simulink model "GaN_Fig5_Clamp_Analog_State"  (R2022b)
settings: Solver=ode15s  StartTime=0.0  StopTime=3e-6  MaxStep=5e-10  RelTol=1e-7  AbsTol=1e-9
model workspace (MAT data in the model file):
  btb_blocking_negative = [0 1e-10 2e-10 3e-10 4e-10 5e-10 6e-10 7e-10 8e-10 9e-10 1e-09 1.1e-09 ... (60002 elements, 30001x2)]
  btb_blocking_positive = [0 1e-10 2e-10 3e-10 4e-10 5e-10 6e-10 7e-10 8e-10 9e-10 1e-09 1.1e-09 ... (60002 elements, 30001x2)]
  btb_improved_negative = [0 1e-10 2e-10 3e-10 4e-10 5e-10 6e-10 7e-10 8e-10 9e-10 1e-09 1.1e-09 ... (60002 elements, 30001x2)]
  btb_improved_positive = [0 1e-10 2e-10 3e-10 4e-10 5e-10 6e-10 7e-10 8e-10 9e-10 1e-09 1.1e-09 ... (60002 elements, 30001x2)]
  dv_blocking_negative = [0 1e-10 2e-10 3e-10 4e-10 5e-10 6e-10 7e-10 8e-10 9e-10 1e-09 1.1e-09 ... (60002 elements, 30001x2)]
  dv_blocking_positive = [0 1e-10 2e-10 3e-10 4e-10 5e-10 6e-10 7e-10 8e-10 9e-10 1e-09 1.1e-09 ... (60002 elements, 30001x2)]
  dv_improved_negative = [0 1e-10 2e-10 3e-10 4e-10 5e-10 6e-10 7e-10 8e-10 9e-10 1e-09 1.1e-09 ... (60002 elements, 30001x2)]
  dv_improved_positive = [0 1e-10 2e-10 3e-10 4e-10 5e-10 6e-10 7e-10 8e-10 9e-10 1e-09 1.1e-09 ... (60002 elements, 30001x2)]
  gb_blocking_negative = [0 1e-10 2e-10 3e-10 4e-10 5e-10 6e-10 7e-10 8e-10 9e-10 1e-09 1.1e-09 ... (60002 elements, 30001x2)]
  gb_blocking_positive = [0 1e-10 2e-10 3e-10 4e-10 5e-10 6e-10 7e-10 8e-10 9e-10 1e-09 1.1e-09 ... (60002 elements, 30001x2)]
  gb_improved_negative = [0 1e-10 2e-10 3e-10 4e-10 5e-10 6e-10 7e-10 8e-10 9e-10 1e-09 1.1e-09 ... (60002 elements, 30001x2)]
  gb_improved_positive = [0 1e-10 2e-10 3e-10 4e-10 5e-10 6e-10 7e-10 8e-10 9e-10 1e-09 1.1e-09 ... (60002 elements, 30001x2)]
  v_blocking_negative = [0 1e-10 2e-10 3e-10 4e-10 5e-10 6e-10 7e-10 8e-10 9e-10 1e-09 1.1e-09 ... (60002 elements, 30001x2)]
  v_blocking_positive = [0 1e-10 2e-10 3e-10 4e-10 5e-10 6e-10 7e-10 8e-10 9e-10 1e-09 1.1e-09 ... (60002 elements, 30001x2)]
  v_improved_negative = [0 1e-10 2e-10 3e-10 4e-10 5e-10 6e-10 7e-10 8e-10 9e-10 1e-09 1.1e-09 ... (60002 elements, 30001x2)]
  v_improved_positive = [0 1e-10 2e-10 3e-10 4e-10 5e-10 6e-10 7e-10 8e-10 9e-10 1e-09 1.1e-09 ... (60002 elements, 30001x2)]
settings Model: Creator=Greatlovers  LastModifiedBy=Greatlovers

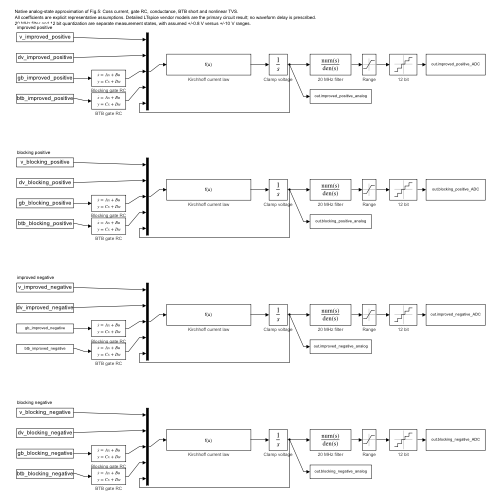
[thumbnail: Simulink's stored preview of the top-level diagram]
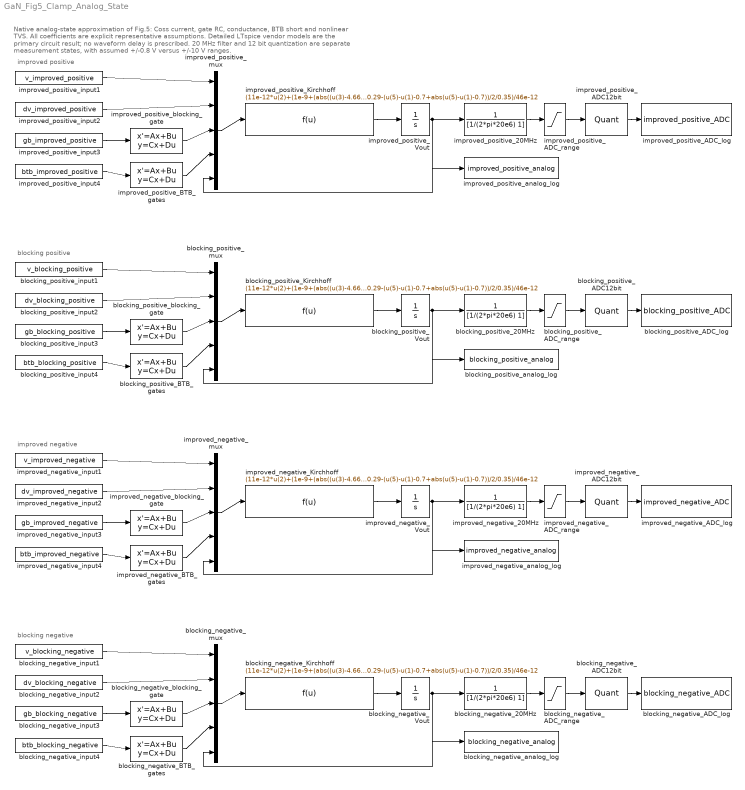
== system GaN_Fig5_Clamp_Analog_State ==
  note: improved positive
  note: blocking positive
  note: improved negative
  note: blocking negative
  note: Native analog-state approximation of Fig.5: Coss current, gate RC, conductance, BTB short and nonlinear TVS.
      | All coefficients are explicit representative assumptions. Detailed LTspice vendor models are the primary circuit result; no waveform delay is prescribed.
      | 20 MHz filter and 12 bit quantization are separate measurement states, with assumed +/-0.8 V versus +/-10 V ranges.
  blocking_negative_20MHz : TransferFcn  Numerator=1  Denominator=[1/(2*pi*20e6) 1]
      settings: AttributesFormatString=20 MHz filter
  blocking_negative_ADC12bit : Quantizer  QuantizationInterval=0.0048828125
      settings: AttributesFormatString=12 bit
  blocking_negative_ADC_log : ToWorkspace  VariableName=blocking_negative_ADC  SaveFormat=Timeseries  SampleTime=-1
  blocking_negative_ADC_range : Saturate  UpperLimit=10  LowerLimit=-10
      settings: AttributesFormatString=Range
  blocking_negative_BTB_gates : StateSpace  A=-1/2.6e-9  B=1/2.6e-9  D=0  InitialCondition=0
      settings: AttributesFormatString=BTB gate RC
  blocking_negative_Kirchhoff : Fcn  Expr=(11e-12*u(2)+(1e-9+(abs((u(3)-4.662)/5.338)-abs((u(3)-4.662)/5.338-1)+1)/2/11)*(u(1)-u(5))-(abs((u(4)-0.6118)/3.8882)-abs((u(4)-0.6118)/3.8882-1)+1)/2/0.122*u(5)-u(5)/1e6-((u(5)-8+abs(u(5)-8))/2-(-u(5)-8+abs(-u(5)-8))/2)/0.29-(u(5)-u(1)-0.7+abs(u(5)-u(1)-0.7))/2/0.35)/46e-12
      settings: AttributesFormatString=Kirchhoff current law
  blocking_negative_Vout : Integrator
      settings: AttributesFormatString=Clamp voltage
  blocking_negative_analog_log : ToWorkspace  VariableName=blocking_negative_analog  SaveFormat=Timeseries  SampleTime=-1
  blocking_negative_blocking_gate : StateSpace  A=-1/1.88e-9  B=1/1.88e-9  D=0  InitialCondition=0
      settings: AttributesFormatString=Blocking gate RC
  blocking_negative_input1 : FromWorkspace  VariableName=v_blocking_negative
  blocking_negative_input2 : FromWorkspace  VariableName=dv_blocking_negative
  blocking_negative_input3 : FromWorkspace  VariableName=gb_blocking_negative
  blocking_negative_input4 : FromWorkspace  VariableName=btb_blocking_negative
  blocking_negative_mux : Mux  Inputs=5
  blocking_positive_20MHz : TransferFcn  Numerator=1  Denominator=[1/(2*pi*20e6) 1]
      settings: AttributesFormatString=20 MHz filter
  blocking_positive_ADC12bit : Quantizer  QuantizationInterval=0.0048828125
      settings: AttributesFormatString=12 bit
  blocking_positive_ADC_log : ToWorkspace  VariableName=blocking_positive_ADC  SaveFormat=Timeseries  SampleTime=-1
  blocking_positive_ADC_range : Saturate  UpperLimit=10  LowerLimit=-10
      settings: AttributesFormatString=Range
  blocking_positive_BTB_gates : StateSpace  A=-1/2.6e-9  B=1/2.6e-9  D=0  InitialCondition=0
      settings: AttributesFormatString=BTB gate RC
  blocking_positive_Kirchhoff : Fcn  Expr=(11e-12*u(2)+(1e-9+(abs((u(3)-4.662)/5.338)-abs((u(3)-4.662)/5.338-1)+1)/2/11)*(u(1)-u(5))-(abs((u(4)-0.6118)/3.8882)-abs((u(4)-0.6118)/3.8882-1)+1)/2/0.122*u(5)-u(5)/1e6-((u(5)-8+abs(u(5)-8))/2-(-u(5)-8+abs(-u(5)-8))/2)/0.29-(u(5)-u(1)-0.7+abs(u(5)-u(1)-0.7))/2/0.35)/46e-12
      settings: AttributesFormatString=Kirchhoff current law
  blocking_positive_Vout : Integrator
      settings: AttributesFormatString=Clamp voltage
  blocking_positive_analog_log : ToWorkspace  VariableName=blocking_positive_analog  SaveFormat=Timeseries  SampleTime=-1
  blocking_positive_blocking_gate : StateSpace  A=-1/1.88e-9  B=1/1.88e-9  D=0  InitialCondition=0
      settings: AttributesFormatString=Blocking gate RC
  blocking_positive_input1 : FromWorkspace  VariableName=v_blocking_positive
  blocking_positive_input2 : FromWorkspace  VariableName=dv_blocking_positive
  blocking_positive_input3 : FromWorkspace  VariableName=gb_blocking_positive
  blocking_positive_input4 : FromWorkspace  VariableName=btb_blocking_positive
  blocking_positive_mux : Mux  Inputs=5
  improved_negative_20MHz : TransferFcn  Numerator=1  Denominator=[1/(2*pi*20e6) 1]
      settings: AttributesFormatString=20 MHz filter
  improved_negative_ADC12bit : Quantizer  QuantizationInterval=0.00039062500000000002
      settings: AttributesFormatString=12 bit
  improved_negative_ADC_log : ToWorkspace  VariableName=improved_negative_ADC  SaveFormat=Timeseries  SampleTime=-1
  improved_negative_ADC_range : Saturate  UpperLimit=0.8  LowerLimit=-0.8
      settings: AttributesFormatString=Range
  improved_negative_BTB_gates : StateSpace  A=-1/2.6e-9  B=1/2.6e-9  D=0  InitialCondition=4.5
      settings: AttributesFormatString=BTB gate RC
  improved_negative_Kirchhoff : Fcn  Expr=(11e-12*u(2)+(1e-9+(abs((u(3)-4.662)/5.338)-abs((u(3)-4.662)/5.338-1)+1)/2/11)*(u(1)-u(5))-(abs((u(4)-0.6118)/3.8882)-abs((u(4)-0.6118)/3.8882-1)+1)/2/0.122*u(5)-u(5)/1e6-((u(5)-8+abs(u(5)-8))/2-(-u(5)-8+abs(-u(5)-8))/2)/0.29-(u(5)-u(1)-0.7+abs(u(5)-u(1)-0.7))/2/0.35)/46e-12
      settings: AttributesFormatString=Kirchhoff current law
  improved_negative_Vout : Integrator
      settings: AttributesFormatString=Clamp voltage
  improved_negative_analog_log : ToWorkspace  VariableName=improved_negative_analog  SaveFormat=Timeseries  SampleTime=-1
  improved_negative_blocking_gate : StateSpace  A=-1/1.88e-9  B=1/1.88e-9  D=0  InitialCondition=0
      settings: AttributesFormatString=Blocking gate RC
  improved_negative_input1 : FromWorkspace  VariableName=v_improved_negative
  improved_negative_input2 : FromWorkspace  VariableName=dv_improved_negative
  improved_negative_input3 : FromWorkspace  VariableName=gb_improved_negative
  improved_negative_input4 : FromWorkspace  VariableName=btb_improved_negative
  improved_negative_mux : Mux  Inputs=5
  improved_positive_20MHz : TransferFcn  Numerator=1  Denominator=[1/(2*pi*20e6) 1]
      settings: AttributesFormatString=20 MHz filter
  improved_positive_ADC12bit : Quantizer  QuantizationInterval=0.00039062500000000002
      settings: AttributesFormatString=12 bit
  improved_positive_ADC_log : ToWorkspace  VariableName=improved_positive_ADC  SaveFormat=Timeseries  SampleTime=-1
  improved_positive_ADC_range : Saturate  UpperLimit=0.8  LowerLimit=-0.8
      settings: AttributesFormatString=Range
  improved_positive_BTB_gates : StateSpace  A=-1/2.6e-9  B=1/2.6e-9  D=0  InitialCondition=4.5
      settings: AttributesFormatString=BTB gate RC
  improved_positive_Kirchhoff : Fcn  Expr=(11e-12*u(2)+(1e-9+(abs((u(3)-4.662)/5.338)-abs((u(3)-4.662)/5.338-1)+1)/2/11)*(u(1)-u(5))-(abs((u(4)-0.6118)/3.8882)-abs((u(4)-0.6118)/3.8882-1)+1)/2/0.122*u(5)-u(5)/1e6-((u(5)-8+abs(u(5)-8))/2-(-u(5)-8+abs(-u(5)-8))/2)/0.29-(u(5)-u(1)-0.7+abs(u(5)-u(1)-0.7))/2/0.35)/46e-12
      settings: AttributesFormatString=Kirchhoff current law
  improved_positive_Vout : Integrator
      settings: AttributesFormatString=Clamp voltage
  improved_positive_analog_log : ToWorkspace  VariableName=improved_positive_analog  SaveFormat=Timeseries  SampleTime=-1
  improved_positive_blocking_gate : StateSpace  A=-1/1.88e-9  B=1/1.88e-9  D=0  InitialCondition=0
      settings: AttributesFormatString=Blocking gate RC
  improved_positive_input1 : FromWorkspace  VariableName=v_improved_positive
  improved_positive_input2 : FromWorkspace  VariableName=dv_improved_positive
  improved_positive_input3 : FromWorkspace  VariableName=gb_improved_positive
  improved_positive_input4 : FromWorkspace  VariableName=btb_improved_positive
  improved_positive_mux : Mux  Inputs=5
  wires:
  improved_positive_input1/1 -> improved_positive_mux/1
  improved_positive_input2/1 -> improved_positive_mux/2
  improved_positive_input3/1 -> improved_positive_blocking_gate/1
  improved_positive_input4/1 -> improved_positive_BTB_gates/1
  improved_positive_blocking_gate/1 -> improved_positive_mux/3
  improved_positive_BTB_gates/1 -> improved_positive_mux/4
  improved_positive_mux/1 -> improved_positive_Kirchhoff/1
  improved_positive_Kirchhoff/1 -> improved_positive_Vout/1
  improved_positive_Vout/1 -> improved_positive_mux/5, improved_positive_20MHz/1, improved_positive_analog_log/1
  improved_positive_20MHz/1 -> improved_positive_ADC_range/1
  improved_positive_ADC_range/1 -> improved_positive_ADC12bit/1
  improved_positive_ADC12bit/1 -> improved_positive_ADC_log/1
  blocking_positive_input1/1 -> blocking_positive_mux/1
  blocking_positive_input2/1 -> blocking_positive_mux/2
  blocking_positive_input3/1 -> blocking_positive_blocking_gate/1
  blocking_positive_input4/1 -> blocking_positive_BTB_gates/1
  blocking_positive_blocking_gate/1 -> blocking_positive_mux/3
  blocking_positive_BTB_gates/1 -> blocking_positive_mux/4
  blocking_positive_mux/1 -> blocking_positive_Kirchhoff/1
  blocking_positive_Kirchhoff/1 -> blocking_positive_Vout/1
  blocking_positive_Vout/1 -> blocking_positive_mux/5, blocking_positive_20MHz/1, blocking_positive_analog_log/1
  blocking_positive_20MHz/1 -> blocking_positive_ADC_range/1
  blocking_positive_ADC_range/1 -> blocking_positive_ADC12bit/1
  blocking_positive_ADC12bit/1 -> blocking_positive_ADC_log/1
  improved_negative_input1/1 -> improved_negative_mux/1
  improved_negative_input2/1 -> improved_negative_mux/2
  improved_negative_input3/1 -> improved_negative_blocking_gate/1
  improved_negative_input4/1 -> improved_negative_BTB_gates/1
  improved_negative_blocking_gate/1 -> improved_negative_mux/3
  improved_negative_BTB_gates/1 -> improved_negative_mux/4
  improved_negative_mux/1 -> improved_negative_Kirchhoff/1
  improved_negative_Kirchhoff/1 -> improved_negative_Vout/1
  improved_negative_Vout/1 -> improved_negative_mux/5, improved_negative_20MHz/1, improved_negative_analog_log/1
  improved_negative_20MHz/1 -> improved_negative_ADC_range/1
  improved_negative_ADC_range/1 -> improved_negative_ADC12bit/1
  improved_negative_ADC12bit/1 -> improved_negative_ADC_log/1
  blocking_negative_input1/1 -> blocking_negative_mux/1
  blocking_negative_input2/1 -> blocking_negative_mux/2
  blocking_negative_input3/1 -> blocking_negative_blocking_gate/1
  blocking_negative_input4/1 -> blocking_negative_BTB_gates/1
  blocking_negative_blocking_gate/1 -> blocking_negative_mux/3
  blocking_negative_BTB_gates/1 -> blocking_negative_mux/4
  blocking_negative_mux/1 -> blocking_negative_Kirchhoff/1
  blocking_negative_Kirchhoff/1 -> blocking_negative_Vout/1
  blocking_negative_Vout/1 -> blocking_negative_mux/5, blocking_negative_20MHz/1, blocking_negative_analog_log/1
  blocking_negative_20MHz/1 -> blocking_negative_ADC_range/1
  blocking_negative_ADC_range/1 -> blocking_negative_ADC12bit/1
  blocking_negative_ADC12bit/1 -> blocking_negative_ADC_log/1
